simulink model "ftbff"  (R2024b)
settings: Solver=VariableStepAuto  StartTime=0.0  StopTime=10.0  RelTol=1e-3
values from neighbouring files (symbols this model uses):
  b = 3    [ftbf.m]
  G = 5    [ftbf.m]
  g = 0.02    [ftbf.m]
  Km = (pi * omega_0) / (10 * G)    (= 2.51327412287)    [ftbf.m]
  Kp = 5    [ftbf.m]
  tau = 0.02    [ftbf.m]
settings Model: Creator=enzoc  LastModifiedBy=enzoc

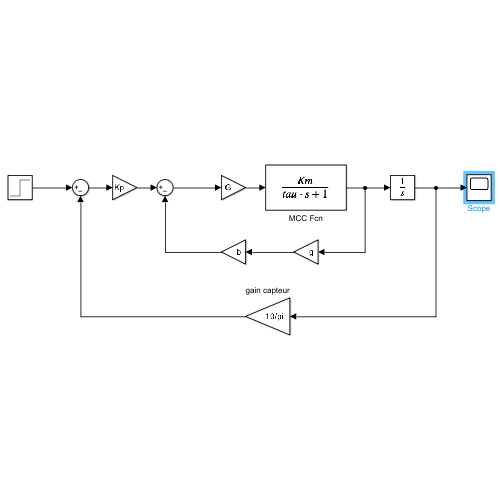
[thumbnail: Simulink's stored preview of the top-level diagram]
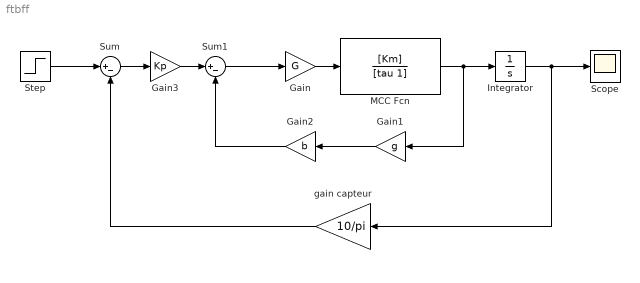
== system ftbff ==
  Gain : Gain  Gain=G
  Gain1 : Gain  Gain=g
  Gain2 : Gain  Gain=b
  Gain3 : Gain  Gain=Kp
  Integrator : Integrator
  MCC Fcn : TransferFcn  Numerator=[Km]  Denominator=[tau 1]
  Scope : Scope
  Step : Step  SampleTime=0
  Sum : Sum  Inputs=|+-
  Sum1 : Sum  Inputs=|+-
  gain capteur : Gain  Gain=10/pi
  wires:
  Gain/1 -> MCC Fcn/1
  MCC Fcn/1 -> Gain1/1, Integrator/1
  Integrator/1 -> gain capteur/1, Scope/1
  gain capteur/1 -> Sum/2
  Step/1 -> Sum/1
  Sum1/1 -> Gain/1
  Sum/1 -> Gain3/1
  Gain1/1 -> Gain2/1
  Gain2/1 -> Sum1/2
  Gain3/1 -> Sum1/1
